simulink model "sm_car_"  (R2026b)
settings: Solver=ode23t  StopTime=100  MaxStep=0.4  AbsTol=1e-3  EnableMultiTasking=on
PreLoadFcn:
  | % Due to usability issue in Repeating Sequence block
  | warning('off','Simulink:Masking:Invalid');
  | 
  | % Eliminate unnecessary warnings in inactive variants
  | % Warnings generated only if you click through inactive variant
  | warning('off','MATLAB:nonExistentField');
  | warning('off','Simulink:Parameters:BlkParamUndefined');
PostLoadFcn:
  | set_param([bdroot '/Vehicle'],'popup_trailer','Off')
  | warning('off','sm:sli:setup:compile:LocalSolverNotSupported')
  | %sm_car_config_maneuver(bdroot,'WOT Braking');
  | sm_car_config_vehicle(bdroot,'false');
  | sm_car_config_logging(bdroot);
InitFcn:
  | sm_car_config_camera;
  | Vehicle = sm_car_vehcfg_checkConfig(Vehicle);
  | sm_car_check_tire_model(bdroot);
StartFcn:
  | tic;
StopFcn:
  | Elapsed_Sim_Time = toc;
  | % disp(['Elapsed Sim Time = ' num2str(Elapsed_Sim_Time)]);
undefined symbols (not defined in the file or in its folder): acc_theta, accel_ramp_rate, Axle1D, AxleIn, Camera, Control, Driver, Init, Maneuver, Pedal, Scene, ShaftL1, ShaftL2, ShaftR1, ShaftR2, Visual, X, xy_data_car_side, Y, Z
libraries: sm_lib x290, fl_lib x171, nesl_utility x144, simulink x60, simulink_extras x14, sdl_lib x14, SimscapeFluids_lib x7, Damper_Element x4, Tire_1x2x x4, ee_lib x3, Scene_Utilities x3, sharedTrackingLibrary x2
(part 12 of 22)

== system sm_car_/Driver/Closed Loop1/Maneuver/PoseTarget Visual/Pace Car ==
  Left Face : sm_lib/Body Elements/Extruded Solid  ExtrusionType=General  PolygonNumSides=3  PolygonOuterRadius=1  PolygonOuterRadiusUnits=m  ExportEntireGeometry=off  ExtrusionCrossSection=xy_data_car_side  ExtrusionCrossSectionUnits=m  ExportConvexHullGeometry=off  ExtrusionLength=thk_side  ExtrusionLengthUnits=m  InertiaType=PointMass  BasedOnType=Density  Density=1000  DensityUnits=kg/m^3  Mass=0  MassUnits=kg  CenterOfMass=[0 0 0]  CenterOfMassUnits=m  MomentsOfInertia=[1 1 1]  MomentsOfInertiaUnits=kg*m^2  ProductsOfInertia=[0 0 0]  ProductsOfInertiaUnits=kg*m^2  GraphicType=FromGeometry  MarkerShape=Sphere  MarkerSize=10  GraphicVisPropType=SimpleVisualProperties  GraphicDiffuseColor=clr_body_geo_left  GraphicOpacity=opc_body_geo_left  GraphicSpecularColor=[0.5 0.5 0.5 1.0]  GraphicAmbientColor=[0.15 0.15 0.15 1.0]  GraphicEmissiveColor=[0.0 0.0 0.0 1.0]  GraphicShininess=75  DoExposeReferenceFrame=on  SerializedFrames=<Frames/>
  Ornament Front : sm_lib/Body Elements/Extruded Solid  ExtrusionType=General  PolygonNumSides=3  PolygonOuterRadius=1  PolygonOuterRadiusUnits=m  ExportEntireGeometry=off  ExtrusionCrossSection=extr_data_emblem_f  ExtrusionCrossSectionUnits=m  ExportConvexHullGeometry=off  ExtrusionLength=0.01  ExtrusionLengthUnits=m  InertiaType=CalculateFromGeometry  BasedOnType=Density  Density=1000  DensityUnits=kg/m^3  Mass=1  MassUnits=kg  CenterOfMass=[0 0 0]  CenterOfMassUnits=m  MomentsOfInertia=[1 1 1]  MomentsOfInertiaUnits=kg*m^2  ProductsOfInertia=[0 0 0]  ProductsOfInertiaUnits=kg*m^2  GraphicType=FromGeometry  MarkerShape=Sphere  MarkerSize=10  GraphicVisPropType=AdvancedVisualProperties  GraphicDiffuseColor=clr_emblem_f  GraphicOpacity=opc_emblem_f  GraphicSpecularColor=[0.5 0.5 0.5 1.0]  GraphicAmbientColor=[0.15 0.15 0.15 1.0]  GraphicEmissiveColor=[clr_emblem_f 1.0]  GraphicShininess=75  DoExposeReferenceFrame=on  SerializedFrames=<Frames/>
  Ornament Rear : sm_lib/Body Elements/Extruded Solid  ExtrusionType=General  PolygonNumSides=3  PolygonOuterRadius=1  PolygonOuterRadiusUnits=m  ExportEntireGeometry=off  ExtrusionCrossSection=extr_data_emblem_r  ExtrusionCrossSectionUnits=m  ExportConvexHullGeometry=off  ExtrusionLength=0.01  ExtrusionLengthUnits=m  InertiaType=CalculateFromGeometry  BasedOnType=Density  Density=1000  DensityUnits=kg/m^3  Mass=1  MassUnits=kg  CenterOfMass=[0 0 0]  CenterOfMassUnits=m  MomentsOfInertia=[1 1 1]  MomentsOfInertiaUnits=kg*m^2  ProductsOfInertia=[0 0 0]  ProductsOfInertiaUnits=kg*m^2  GraphicType=FromGeometry  MarkerShape=Sphere  MarkerSize=10  GraphicVisPropType=SimpleVisualProperties  GraphicDiffuseColor=clr_emblem_r  GraphicOpacity=opc_emblem_r  GraphicSpecularColor=[0.5 0.5 0.5 1.0]  GraphicAmbientColor=[0.15 0.15 0.15 1.0]  GraphicEmissiveColor=[0.0 0.0 0.0 1.0]  GraphicShininess=75  DoExposeReferenceFrame=on  SerializedFrames=<Frames/>
  Rear View : sm_lib/Frames and Transforms/Reference Frame
  Right Face : sm_lib/Body Elements/Extruded Solid  ExtrusionType=General  PolygonNumSides=3  PolygonOuterRadius=1  PolygonOuterRadiusUnits=m  ExportEntireGeometry=off  ExtrusionCrossSection=xy_data_car_side  ExtrusionCrossSectionUnits=m  ExportConvexHullGeometry=off  ExtrusionLength=thk_side  ExtrusionLengthUnits=m  InertiaType=PointMass  BasedOnType=Density  Density=1000  DensityUnits=kg/m^3  Mass=0  MassUnits=kg  CenterOfMass=[0 0 0]  CenterOfMassUnits=m  MomentsOfInertia=[1 1 1]  MomentsOfInertiaUnits=kg*m^2  ProductsOfInertia=[0 0 0]  ProductsOfInertiaUnits=kg*m^2  GraphicType=FromGeometry  MarkerShape=Sphere  MarkerSize=10  GraphicVisPropType=SimpleVisualProperties  GraphicDiffuseColor=clr_body_geo_right  GraphicOpacity=opc_body_geo_right  GraphicSpecularColor=[0.5 0.5 0.5 1.0]  GraphicAmbientColor=[0.15 0.15 0.15 1.0]  GraphicEmissiveColor=[0.0 0.0 0.0 1.0]  GraphicShininess=75  DoExposeReferenceFrame=on  SerializedFrames=<Frames/>
  Top Surface : sm_lib/Body Elements/Extruded Solid  ExtrusionType=General  PolygonNumSides=3  PolygonOuterRadius=1  PolygonOuterRadiusUnits=m  ExportEntireGeometry=off  ExtrusionCrossSection=xy_data_car_top  ExtrusionCrossSectionUnits=m  ExportConvexHullGeometry=off  ExtrusionLength=car_track  ExtrusionLengthUnits=m  InertiaType=PointMass  BasedOnType=Density  Density=0  DensityUnits=kg/m^3  Mass=0  MassUnits=kg  CenterOfMass=[0 0 0]  CenterOfMassUnits=m  MomentsOfInertia=[1 1 1]  MomentsOfInertiaUnits=kg*m^2  ProductsOfInertia=[0 0 0]  ProductsOfInertiaUnits=kg*m^2  GraphicType=FromGeometry  MarkerShape=Sphere  MarkerSize=10  GraphicVisPropType=SimpleVisualProperties  GraphicDiffuseColor=clr_body_geo_top  GraphicOpacity=opc_body_geo_top  GraphicSpecularColor=[0.5 0.5 0.5 1.0]  GraphicAmbientColor=[0.15 0.15 0.15 1.0]  GraphicEmissiveColor=[0.0 0.0 0.0 1.0]  GraphicShininess=75  DoExposeReferenceFrame=on  SerializedFrames=<Frames/>
  Transform Extrusion Axes : sm_lib/Frames and Transforms/Rigid Transform  RotationMethod=StandardAxis  FollAlignAxisA=+X  BaseAlignAxisA=+Y  FollAlignAxisB=+Y  BaseAlignAxisB=+Z  RotationStandardAxis=+X  RotationAngle=90  RotationAngleUnits=deg  RotationArbitraryAxis=[0 0 1]  RotationSequenceAxes=FollowerAxes  RotationSequence=XYX  RotationSequenceAngles=[0 0 0]  RotationSequenceAnglesUnits=deg  RotationMatrix=[1 0 0; 0 1 0; 0 0 1]  Quaternion=[1 0 0 0]  TranslationMethod=None  TranslationCartesianOffset=[0 0 0]  TranslationCartesianOffsetUnits=m  TranslationStandardAxis=+Z  TranslationStandardOffset=0  TranslationStandardOffsetUnits=m  TranslationROffset=0  TranslationROffsetUnits=m  TranslationThetaOffset=0  TranslationThetaOffsetUnits=deg  TranslationZOffset=0  TranslationZOffsetUnits=m
  Transform Ornament Front : sm_lib/Frames and Transforms/Rigid Transform  RotationMethod=RotationSequence  FollAlignAxisA=+X  BaseAlignAxisA=+Y  FollAlignAxisB=+Y  BaseAlignAxisB=+Z  RotationStandardAxis=+Z  RotationAngle=90  RotationAngleUnits=deg  RotationArbitraryAxis=[0 0 1]  RotationSequenceAxes=FollowerAxes  RotationSequence=ZXY  RotationSequenceAngles=[90 90 0]  RotationSequenceAnglesUnits=deg  RotationMatrix=[1 0 0; 0 1 0; 0 0 1]  Quaternion=[1 0 0 0]  TranslationMethod=Cartesian  TranslationCartesianOffset=[max(xy_data_car_side(:,1)) 0 min(xy_data_car_side(:,2))+0.15]  TranslationCartesianOffsetUnits=m  TranslationStandardAxis=+Z  TranslationStandardOffset=1  TranslationStandardOffsetUnits=m  TranslationROffset=0  TranslationROffsetUnits=m  TranslationThetaOffset=0  TranslationThetaOffsetUnits=deg  TranslationZOffset=0  TranslationZOffsetUnits=m
  Transform Ornament Rear : sm_lib/Frames and Transforms/Rigid Transform  RotationMethod=RotationSequence  FollAlignAxisA=+X  BaseAlignAxisA=+Y  FollAlignAxisB=+Y  BaseAlignAxisB=+Z  RotationStandardAxis=+Z  RotationAngle=90  RotationAngleUnits=deg  RotationArbitraryAxis=[0 0 1]  RotationSequenceAxes=FollowerAxes  RotationSequence=ZXY  RotationSequenceAngles=[90 90 180]  RotationSequenceAnglesUnits=deg  RotationMatrix=[1 0 0; 0 1 0; 0 0 1]  Quaternion=[1 0 0 0]  TranslationMethod=Cartesian  TranslationCartesianOffset=[min(xy_data_car_side(:,1))+0.1 0 min(xy_data_car_side(:,2))+0.15]  TranslationCartesianOffsetUnits=m  TranslationStandardAxis=+Z  TranslationStandardOffset=1  TranslationStandardOffsetUnits=m  TranslationROffset=0  TranslationROffsetUnits=m  TranslationThetaOffset=0  TranslationThetaOffsetUnits=deg  TranslationZOffset=0  TranslationZOffsetUnits=m
  Transform Rear View : sm_lib/Frames and Transforms/Rigid Transform  RotationMethod=None  FollAlignAxisA=+X  BaseAlignAxisA=+Y  FollAlignAxisB=+Y  BaseAlignAxisB=+Z  RotationStandardAxis=+Z  RotationAngle=0.0  RotationAngleUnits=deg  RotationArbitraryAxis=[0 0 1]  RotationSequenceAxes=FollowerAxes  RotationSequence=XYX  RotationSequenceAngles=[0 0 0]  RotationSequenceAnglesUnits=deg  RotationMatrix=[1 0 0; 0 1 0; 0 0 1]  Quaternion=[1 0 0 0]  TranslationMethod=Cartesian  TranslationCartesianOffset=[min(xy_data_car_side(:,1))-4 0 min(xy_data_car_side(:,2))+1]  TranslationCartesianOffsetUnits=m  TranslationStandardAxis=+Z  TranslationStandardOffset=0  TranslationStandardOffsetUnits=m  TranslationROffset=0  TranslationROffsetUnits=m  TranslationThetaOffset=0  TranslationThetaOffsetUnits=deg  TranslationZOffset=0  TranslationZOffsetUnits=m
  Transform Reference : sm_lib/Frames and Transforms/Rigid Transform  RotationMethod=None  FollAlignAxisA=+X  BaseAlignAxisA=+Y  FollAlignAxisB=+Y  BaseAlignAxisB=+Z  RotationStandardAxis=+Z  RotationAngle=0.0  RotationAngleUnits=deg  RotationArbitraryAxis=[0 0 1]  RotationSequenceAxes=FollowerAxes  RotationSequence=XYX  RotationSequenceAngles=[0 0 0]  RotationSequenceAnglesUnits=deg  RotationMatrix=[1 0 0; 0 1 0; 0 0 1]  Quaternion=[1 0 0 0]  TranslationMethod=Cartesian  TranslationCartesianOffset=offset_ref  TranslationCartesianOffsetUnits=m  TranslationStandardAxis=+Z  TranslationStandardOffset=0  TranslationStandardOffsetUnits=m  TranslationROffset=0  TranslationROffsetUnits=m  TranslationThetaOffset=0  TranslationThetaOffsetUnits=deg  TranslationZOffset=0  TranslationZOffsetUnits=m
  Transform Left Face : sm_lib/Frames and Transforms/Rigid Transform  RotationMethod=None  FollAlignAxisA=+X  BaseAlignAxisA=+Y  FollAlignAxisB=+Y  BaseAlignAxisB=+Z  RotationStandardAxis=+Z  RotationAngle=0.0  RotationAngleUnits=deg  RotationArbitraryAxis=[0 0 1]  RotationSequenceAxes=FollowerAxes  RotationSequence=XYX  RotationSequenceAngles=[0 0 0]  RotationSequenceAnglesUnits=deg  RotationMatrix=[1 0 0; 0 1 0; 0 0 1]  Quaternion=[1 0 0 0]  TranslationMethod=StandardAxis  TranslationCartesianOffset=[0 0 0]  TranslationCartesianOffsetUnits=m  TranslationStandardAxis=-Z  TranslationStandardOffset=car_track/2-thk_side/2  TranslationStandardOffsetUnits=m  TranslationROffset=0  TranslationROffsetUnits=m  TranslationThetaOffset=0  TranslationThetaOffsetUnits=deg  TranslationZOffset=0  TranslationZOffsetUnits=m
  Transform Right Face : sm_lib/Frames and Transforms/Rigid Transform  RotationMethod=None  FollAlignAxisA=+X  BaseAlignAxisA=+Y  FollAlignAxisB=+Y  BaseAlignAxisB=+Z  RotationStandardAxis=+Z  RotationAngle=0.0  RotationAngleUnits=deg  RotationArbitraryAxis=[0 0 1]  RotationSequenceAxes=FollowerAxes  RotationSequence=XYX  RotationSequenceAngles=[0 0 0]  RotationSequenceAnglesUnits=deg  RotationMatrix=[1 0 0; 0 1 0; 0 0 1]  Quaternion=[1 0 0 0]  TranslationMethod=StandardAxis  TranslationCartesianOffset=[0 0 0]  TranslationCartesianOffsetUnits=m  TranslationStandardAxis=+Z  TranslationStandardOffset=car_track/2-thk_side/2  TranslationStandardOffsetUnits=m  TranslationROffset=0  TranslationROffsetUnits=m  TranslationThetaOffset=0  TranslationThetaOffsetUnits=deg  TranslationZOffset=0  TranslationZOffsetUnits=m
  FA : PMIOPort  Side=Right
  P : PMIOPort  Port=2  Side=Left
  connections:
  Transform Reference/LConn1 -- P/RConn1 -- FA/RConn1
  Transform Rear View/RConn1 -- Rear View/RConn1
  Transform Reference/RConn1 -- Transform Ornament Front/LConn1 -- Transform Ornament Rear/LConn1 -- Transform Rear View/LConn1 -- Transform Extrusion Axes/LConn1
  Left Face/RConn1 -- Transform Left Face/RConn1
  Transform Extrusion Axes/RConn1 -- Transform Right Face/LConn1 -- Top Surface/RConn1 -- Transform Left Face/LConn1
  Right Face/RConn1 -- Transform Right Face/RConn1
  Transform Ornament Front/RConn1 -- Ornament Front/RConn1
  Transform Ornament Rear/RConn1 -- Ornament Rear/RConn1

== system sm_car_/Vehicle/Vehicle/Brakes/PedalAbstract DiscDisc/Actuator L1 ==
  Pedal : Inport
  Filter : TransferFcn  Numerator=brk_max_p  Denominator=[brk_filt 1]
  Simulink-PS Converter : nesl_utility/Simulink-PS Converter  PhysicalDomain=network_engine_domain  SubClassName=ps_input  LeftPortType=input  RightPortType=output  PseudoPeriodic=off  Frequencies=[]  NoiseDistribution=none  NoiseParameters=[]  Unit=1  AffineConversion=off  FilteringAndDerivatives=provide  SimscapeFilterOrder=1  InputFilterTimeConstant=0.001  UdotUserProvided=0
  P : PMIOPort  Side=Right
  wires:
  Pedal/1 -> Filter/1
  Filter/1 -> Simulink-PS Converter/1
  connections:
  Simulink-PS Converter/RConn1 -- P/RConn1

== system sm_car_/Vehicle/Vehicle/Brakes/PedalAbstract DiscDisc/Actuator L2 ==
  Pedal : Inport
  Filter : TransferFcn  Numerator=brk_max_p  Denominator=[brk_filt 1]
  Simulink-PS Converter : nesl_utility/Simulink-PS Converter  PhysicalDomain=network_engine_domain  SubClassName=ps_input  LeftPortType=input  RightPortType=output  PseudoPeriodic=off  Frequencies=[]  NoiseDistribution=none  NoiseParameters=[]  Unit=1  AffineConversion=off  FilteringAndDerivatives=provide  SimscapeFilterOrder=1  InputFilterTimeConstant=0.001  UdotUserProvided=0
  P : PMIOPort  Side=Right
  wires:
  Pedal/1 -> Filter/1
  Filter/1 -> Simulink-PS Converter/1
  connections:
  Simulink-PS Converter/RConn1 -- P/RConn1

== system sm_car_/Vehicle/Vehicle/Brakes/PedalAbstract DiscDisc/Actuator R1 ==
  Pedal : Inport
  Filter : TransferFcn  Numerator=brk_max_p  Denominator=[brk_filt 1]
  Simulink-PS Converter : nesl_utility/Simulink-PS Converter  PhysicalDomain=network_engine_domain  SubClassName=ps_input  LeftPortType=input  RightPortType=output  PseudoPeriodic=off  Frequencies=[]  NoiseDistribution=none  NoiseParameters=[]  Unit=1  AffineConversion=off  FilteringAndDerivatives=provide  SimscapeFilterOrder=1  InputFilterTimeConstant=0.001  UdotUserProvided=0
  P : PMIOPort  Side=Right
  wires:
  Pedal/1 -> Filter/1
  Filter/1 -> Simulink-PS Converter/1
  connections:
  Simulink-PS Converter/RConn1 -- P/RConn1

== system sm_car_/Vehicle/Vehicle/Brakes/PedalAbstract DiscDisc/Actuator R2 ==
  Pedal : Inport
  Filter : TransferFcn  Numerator=brk_max_p  Denominator=[brk_filt 1]
  Simulink-PS Converter : nesl_utility/Simulink-PS Converter  PhysicalDomain=network_engine_domain  SubClassName=ps_input  LeftPortType=input  RightPortType=output  PseudoPeriodic=off  Frequencies=[]  NoiseDistribution=none  NoiseParameters=[]  Unit=1  AffineConversion=off  FilteringAndDerivatives=provide  SimscapeFilterOrder=1  InputFilterTimeConstant=0.001  UdotUserProvided=0
  P : PMIOPort  Side=Right
  wires:
  Pedal/1 -> Filter/1
  Filter/1 -> Simulink-PS Converter/1
  connections:
  Simulink-PS Converter/RConn1 -- P/RConn1

== system sm_car_/Vehicle/Vehicle/Brakes/PedalAbstract DiscDisc/Sensing Torque L1 ==
  Ideal Torque Sensor : fl_lib/Mechanical/Mechanical Sensors/Ideal Torque Sensor
  PS-Simulink Converter : nesl_utility/PS-Simulink Converter  PhysicalDomain=network_engine_domain  SubClassName=ps_output  LeftPortType=input  RightPortType=output  PseudoPeriodic=off  Frequencies=[]  VectorFormat=1-D array  Unit=N*m  AffineConversion=off
  C : PMIOPort  Side=Right
  R : PMIOPort  Port=2  Side=Left
  T : Outport  VectorParamsAs1DForOutWhenUnconnected=off
  wires:
  PS-Simulink Converter/1 -> T/1
  connections:
  PS-Simulink Converter/LConn1 -- Ideal Torque Sensor/RConn2
  Ideal Torque Sensor/RConn1 -- C/RConn1
  Ideal Torque Sensor/LConn1 -- R/RConn1

== system sm_car_/Vehicle/Vehicle/Brakes/PedalAbstract DiscDisc/Sensing Torque L2 ==
  Ideal Torque Sensor : fl_lib/Mechanical/Mechanical Sensors/Ideal Torque Sensor
  PS-Simulink Converter : nesl_utility/PS-Simulink Converter  PhysicalDomain=network_engine_domain  SubClassName=ps_output  LeftPortType=input  RightPortType=output  PseudoPeriodic=off  Frequencies=[]  VectorFormat=1-D array  Unit=N*m  AffineConversion=off
  C : PMIOPort  Side=Right
  R : PMIOPort  Port=2  Side=Left
  T : Outport  VectorParamsAs1DForOutWhenUnconnected=off
  wires:
  PS-Simulink Converter/1 -> T/1
  connections:
  PS-Simulink Converter/LConn1 -- Ideal Torque Sensor/RConn2
  Ideal Torque Sensor/RConn1 -- C/RConn1
  Ideal Torque Sensor/LConn1 -- R/RConn1

== system sm_car_/Vehicle/Vehicle/Brakes/PedalAbstract DiscDisc/Sensing Torque R1 ==
  Ideal Torque Sensor : fl_lib/Mechanical/Mechanical Sensors/Ideal Torque Sensor
  PS-Simulink Converter : nesl_utility/PS-Simulink Converter  PhysicalDomain=network_engine_domain  SubClassName=ps_output  LeftPortType=input  RightPortType=output  PseudoPeriodic=off  Frequencies=[]  VectorFormat=1-D array  Unit=N*m  AffineConversion=off
  C : PMIOPort  Side=Right
  R : PMIOPort  Port=2  Side=Left
  T : Outport  VectorParamsAs1DForOutWhenUnconnected=off
  wires:
  PS-Simulink Converter/1 -> T/1
  connections:
  Ideal Torque Sensor/LConn1 -- R/RConn1
  Ideal Torque Sensor/RConn1 -- C/RConn1
  PS-Simulink Converter/LConn1 -- Ideal Torque Sensor/RConn2

== system sm_car_/Vehicle/Vehicle/Brakes/PedalAbstract DiscDisc/Sensing Torque R2 ==
  Ideal Torque Sensor : fl_lib/Mechanical/Mechanical Sensors/Ideal Torque Sensor
  PS-Simulink Converter : nesl_utility/PS-Simulink Converter  PhysicalDomain=network_engine_domain  SubClassName=ps_output  LeftPortType=input  RightPortType=output  PseudoPeriodic=off  Frequencies=[]  VectorFormat=1-D array  Unit=N*m  AffineConversion=off
  C : PMIOPort  Side=Right
  R : PMIOPort  Port=2  Side=Left
  T : Outport  VectorParamsAs1DForOutWhenUnconnected=off
  wires:
  PS-Simulink Converter/1 -> T/1
  connections:
  Ideal Torque Sensor/LConn1 -- R/RConn1
  Ideal Torque Sensor/RConn1 -- C/RConn1
  PS-Simulink Converter/LConn1 -- Ideal Torque Sensor/RConn2

== system sm_car_/Vehicle/Vehicle/Chassis/Aero/Subsystem ==
  RdBus : Inport
  Actuator dynamics : Subsystem  mask(First-order lag supporting vector signals){b=0.5, x_initial=0}
      mask prompts: b "Filter time constant"; x_initial "Initial output"
      mask help: Models a lag of the form 1/(b*s+1) where s is the Laplace operator.
  Bus Selector : BusSelector  OutputSignals=fx,fy,fz
  Mux : Mux  Inputs=3
  Simulink-PS Converter : nesl_utility/Simulink-PS Converter  PhysicalDomain=network_engine_domain  SubClassName=ps_input  LeftPortType=input  RightPortType=output  PseudoPeriodic=off  Frequencies=[]  NoiseDistribution=none  NoiseParameters=[]  Unit=1  AffineConversion=off  FilteringAndDerivatives=provide  SimscapeFilterOrder=1  InputFilterTimeConstant=0.001  UdotUserProvided=0
  fWind : PMIOPort  Side=Right
  wires:
  Actuator dynamics/1(Out) -> Simulink-PS Converter/1
  RdBus/1 -> Bus Selector/1
  Bus Selector/3 -> Mux/3  "<fz>"
  Bus Selector/2 -> Mux/2  "<fy>"
  Bus Selector/1 -> Mux/1  "<fx>"
  Mux/1 -> Actuator dynamics/1(In)
  connections:
  Simulink-PS Converter/RConn1 -- fWind/RConn1

== system sm_car_/Vehicle/Vehicle/Chassis/Body/Body Geometry ==
  CAD FSAE Achilles : Subsystem  VariantControl=CAD_FSAE_Achilles  mask(FSAE Body Geometry){body_offset=BodyGeometry.sOffset.Value, body_orient=BodyGeometry.aOffset.Value, body_clr=BodyGeometry.Color.Value, body_opc=BodyGeometry.Opacity.Value, aero_clr=BodyGeometry.AeroColor.Value, aero_opc=BodyGeometry.AeroOpacity.Value, extr_data_emblem_aero=Visual.PaceCar.emblem.data*0.3, extr_data_emblem_hood=Visual.PaceCar.emblem.data*0.3, clr_emblem_aero=Visual.clr.orange, clr_emblem_hood=Visual.clr.orange, opc_emblem_aero=Visual.emblem.opc, opc_emblem_hood=Visual.emblem.opc}
      mask prompts: body_offset "Body Offset [x y z] (m)"; body_orient "Body Orientation [R P Y] (rad)"; body_clr "Body Color [R G B] (0-1)"; body_opc "Body Opacity (0-1)"; aero_clr "Aero Color [R G B] (0-1)"; aero_opc "Aero Opacity (0-1)"; extr_data_emblem_aero "Emblem Data Aero [xy] (m)"; extr_data_emblem_hood "Emblem Data Hood [xy] (m)"; clr_emblem_aero "Emblem Color Aero [R G B] (0-1)"; clr_emblem_hood "Emblem Color Hood [R G B] (0-1)"; opc_emblem_aero "Emblem Opacity Aero (0-1)"; opc_emblem_hood "Emblem Opacity Hood (0-1)"
      mask help: CAD geometry of Formula Student Vehicle.
      mask TypeOptions extr_data_emblem_aero:
      | Aero/Ornament
      | Left/ExtrusionCrossSection | Aero/Ornament
      | Right/ExtrusionCrossSection
      mask TypeOptions extr_data_emblem_hood:
      | Body/Ornament
      | Hood/ExtrusionCrossSection
      mask TypeOptions clr_emblem_aero:
      | Aero/Ornament
      | Left/GraphicDiffuseColor | Aero/Ornament
      | Right/GraphicDiffuseColor
      mask TypeOptions clr_emblem_hood:
      | Body/Ornament
      | Hood/GraphicDiffuseColor
      mask TypeOptions opc_emblem_aero:
      | Aero/Ornament
      | Left/GraphicOpacity | Aero/Ornament
      | Right/GraphicOpacity
      mask TypeOptions opc_emblem_hood:
      | Body/Ornament
      | Hood/GraphicOpacity
      mask DialogControl cont_emblem Prompt: Emblem
      mask Display: image('sm_car_bodygeometry_cad_fsae_achilles.png');
  FA : PMIOPort  Side=Right
  P : PMIOPort  Port=2  Side=Left

== system sm_car_/Vehicle/Vehicle/Chassis/Body/Body Load ==
  None : Subsystem  VariantControl=None
  " FA" : PMIOPort  Side=Left

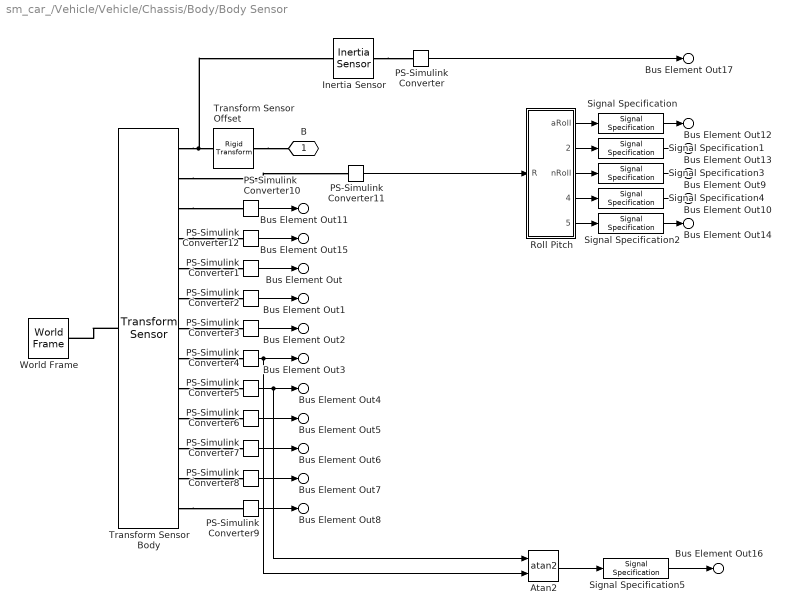
== system sm_car_/Vehicle/Vehicle/Chassis/Body/Body Sensor ==
  Atan2 : Trigonometry  Operator=atan2
  Inertia Sensor : sm_lib/Body Elements/Inertia Sensor  SensorExtent=Mechanism  SpanWeldJoints=off  ExcludeGroundedBodies=on  MeasurementFrame=Attached  SenseMass=off  SenseCenterOfMass=off  SenseInertiaMatrix=off  SenseCenteredInertiaMatrix=on  SensePrincipalInertiaMatrix=off  SenseRotationMatrix=off  GraphicType=PrincipalInertiaFrame  PrincipalInertiaFrameSize=20  GraphicVisPropType=SimpleVisualProperties  GraphicDiffuseColor=[0.5 0.5 0.5]  GraphicOpacity=1  GraphicSpecularColor=[0.5 0.5 0.5 1.0]  GraphicAmbientColor=[0.15 0.15 0.15 1.0]  GraphicEmissiveColor=[0.0 0.0 0.0 1.0]  GraphicShininess=75
  PS-Simulink Converter : nesl_utility/PS-Simulink Converter  PhysicalDomain=network_engine_domain  SubClassName=ps_output  LeftPortType=input  RightPortType=output  PseudoPeriodic=off  Frequencies=[]  VectorFormat=inherit  Unit=kg*m^2  AffineConversion=off
  PS-Simulink Converter1 : nesl_utility/PS-Simulink Converter  PhysicalDomain=network_engine_domain  SubClassName=ps_output  LeftPortType=input  RightPortType=output  PseudoPeriodic=off  Frequencies=[]  VectorFormat=1-D array  Unit=m  AffineConversion=off
  PS-Simulink Converter10 : nesl_utility/PS-Simulink Converter  PhysicalDomain=network_engine_domain  SubClassName=ps_output  LeftPortType=input  RightPortType=output  PseudoPeriodic=off  Frequencies=[]  VectorFormat=inherit  Unit=rad/s  AffineConversion=off
  PS-Simulink Converter11 : nesl_utility/PS-Simulink Converter  PhysicalDomain=network_engine_domain  SubClassName=ps_output  LeftPortType=input  RightPortType=output  PseudoPeriodic=off  Frequencies=[]  VectorFormat=1-D array  Unit=1  AffineConversion=off
  PS-Simulink Converter12 : nesl_utility/PS-Simulink Converter  PhysicalDomain=network_engine_domain  SubClassName=ps_output  LeftPortType=input  RightPortType=output  PseudoPeriodic=off  Frequencies=[]  VectorFormat=inherit  Unit=rad/s^2  AffineConversion=off
  PS-Simulink Converter2 : nesl_utility/PS-Simulink Converter  PhysicalDomain=network_engine_domain  SubClassName=ps_output  LeftPortType=input  RightPortType=output  PseudoPeriodic=off  Frequencies=[]  VectorFormat=1-D array  Unit=m  AffineConversion=off
  PS-Simulink Converter3 : nesl_utility/PS-Simulink Converter  PhysicalDomain=network_engine_domain  SubClassName=ps_output  LeftPortType=input  RightPortType=output  PseudoPeriodic=off  Frequencies=[]  VectorFormat=1-D array  Unit=m  AffineConversion=off
  PS-Simulink Converter4 : nesl_utility/PS-Simulink Converter  PhysicalDomain=network_engine_domain  SubClassName=ps_output  LeftPortType=input  RightPortType=output  PseudoPeriodic=off  Frequencies=[]  VectorFormat=1-D array  Unit=m/s  AffineConversion=off
  PS-Simulink Converter5 : nesl_utility/PS-Simulink Converter  PhysicalDomain=network_engine_domain  SubClassName=ps_output  LeftPortType=input  RightPortType=output  PseudoPeriodic=off  Frequencies=[]  VectorFormat=1-D array  Unit=m/s  AffineConversion=off
  PS-Simulink Converter6 : nesl_utility/PS-Simulink Converter  PhysicalDomain=network_engine_domain  SubClassName=ps_output  LeftPortType=input  RightPortType=output  PseudoPeriodic=off  Frequencies=[]  VectorFormat=1-D array  Unit=m/s  AffineConversion=off
  PS-Simulink Converter7 : nesl_utility/PS-Simulink Converter  PhysicalDomain=network_engine_domain  SubClassName=ps_output  LeftPortType=input  RightPortType=output  PseudoPeriodic=off  Frequencies=[]  VectorFormat=1-D array  Unit=m/s^2  AffineConversion=off
  PS-Simulink Converter8 : nesl_utility/PS-Simulink Converter  PhysicalDomain=network_engine_domain  SubClassName=ps_output  LeftPortType=input  RightPortType=output  PseudoPeriodic=off  Frequencies=[]  VectorFormat=1-D array  Unit=m/s^2  AffineConversion=off
  PS-Simulink Converter9 : nesl_utility/PS-Simulink Converter  PhysicalDomain=network_engine_domain  SubClassName=ps_output  LeftPortType=input  RightPortType=output  PseudoPeriodic=off  Frequencies=[]  VectorFormat=1-D array  Unit=m/s^2  AffineConversion=off
  Roll Pitch : Subsystem
  Signal Specification{,1..2,5} (4 alike) : SignalSpecification  Unit=rad
  Signal Specification3 : SignalSpecification  Unit=rad/s
  Signal Specification4 : SignalSpecification  Unit=rad/s
  Transform Sensor Offset : sm_lib/Frames and Transforms/Rigid Transform  RotationMethod=None  FollAlignAxisA=+X  BaseAlignAxisA=+Y  FollAlignAxisB=+Y  BaseAlignAxisB=+Z  RotationStandardAxis=+Z  RotationAngle=0.0  RotationAngleUnits=deg  RotationArbitraryAxis=[0 0 1]  RotationSequenceAxes=FollowerAxes  RotationSequence=XYX  RotationSequenceAngles=[0 0 0]  RotationSequenceAnglesUnits=deg  RotationMatrix=[1 0 0; 0 1 0; 0 0 1]  Quaternion=[1 0 0 0]  TranslationMethod=Cartesian  TranslationCartesianOffset=offset_body_sensor  TranslationCartesianOffsetUnits=m  TranslationStandardAxis=+Z  TranslationStandardOffset=0  TranslationStandardOffsetUnits=m  TranslationROffset=0  TranslationROffsetUnits=m  TranslationThetaOffset=0  TranslationThetaOffsetUnits=deg  TranslationZOffset=0  TranslationZOffsetUnits=m
  Transform Sensor Body : sm_lib/Frames and Transforms/Transform Sensor  ObservationFrame=World  ExpressedInFrame=Follower  RotationSequence=XYX  SenseAngle=off  SenseAxis=off  SenseQ=off  SenseR=on  SenseRotationSequence=off  SenseOmegaX=off  SenseOmegaY=off  SenseOmegaZ=on  SenseOmega=off  SenseQDot=off  SenseRDot=off  SenseRotationSequenceDot=off  SenseAlphaX=off  SenseAlphaY=off  SenseAlphaZ=on  SenseAlpha=off  SenseQDDot=off  SenseRDDot=off  SenseX=on  SenseY=on  SenseZ=on  SenseXYZ=off  SenseRad=off  SenseAzim=off  SenseDist=off  SenseInc=off  SenseXDot=on  SenseYDot=on  SenseZDot=on  SenseXYZDot=off  SenseRadDot=off  SenseAzimDot=off  SenseDistDot=off  SenseIncDot=off  SenseXDDot=on  SenseYDDot=on  SenseZDDot=on  SenseXYZDDot=off  SenseRadDDot=off  SenseAzimDDot=off  SenseDistDDot=off  SenseIncDDot=off
  World Frame : sm_lib/Frames and Transforms/World Frame
  B : PMIOPort  Side=Left
  Bus Element Out : Outport  VectorParamsAs1DForOutWhenUnconnected=off  PortName=Body  Element=x
  Bus Element Out1 : Outport  VectorParamsAs1DForOutWhenUnconnected=off  PortName=Body  Element=y
  Bus Element Out2 : Outport  VectorParamsAs1DForOutWhenUnconnected=off  PortName=Body  Element=z
  Bus Element Out3 : Outport  VectorParamsAs1DForOutWhenUnconnected=off  PortName=Body  Element=vx
  Bus Element Out4 : Outport  VectorParamsAs1DForOutWhenUnconnected=off  PortName=Body  Element=vy
  Bus Element Out5 : Outport  VectorParamsAs1DForOutWhenUnconnected=off  PortName=Body  Element=vz
  Bus Element Out6 : Outport  VectorParamsAs1DForOutWhenUnconnected=off  PortName=Body  Element=gx
  Bus Element Out7 : Outport  VectorParamsAs1DForOutWhenUnconnected=off  PortName=Body  Element=gy
  Bus Element Out8 : Outport  VectorParamsAs1DForOutWhenUnconnected=off  PortName=Body  Element=gz
  Bus Element Out9 : Outport  VectorParamsAs1DForOutWhenUnconnected=off  PortName=Body  Element=nRoll
  Bus Element Out10 : Outport  VectorParamsAs1DForOutWhenUnconnected=off  PortName=Body  Element=nPitch
  Bus Element Out11 : Outport  VectorParamsAs1DForOutWhenUnconnected=off  PortName=Body  Element=nYaw
  Bus Element Out12 : Outport  VectorParamsAs1DForOutWhenUnconnected=off  PortName=Body  Element=aRoll
  Bus Element Out13 : Outport  VectorParamsAs1DForOutWhenUnconnected=off  PortName=Body  Element=aPitch
  Bus Element Out14 : Outport  VectorParamsAs1DForOutWhenUnconnected=off  PortName=Body  Element=aYaw
  Bus Element Out15 : Outport  VectorParamsAs1DForOutWhenUnconnected=off  PortName=Body  Element=gYaw
  Bus Element Out16 : Outport  VectorParamsAs1DForOutWhenUnconnected=off  PortName=Body  Element=aSideSlip
  Bus Element Out17 : Outport  VectorParamsAs1DForOutWhenUnconnected=off  PortName=Body  Element=InertiaMatrix
  wires:
  PS-Simulink Converter9/1 -> Bus Element Out8/1
  PS-Simulink Converter11/1 -> Roll Pitch/1(R)
  PS-Simulink Converter6/1 -> Bus Element Out5/1
  PS-Simulink Converter7/1 -> Bus Element Out6/1
  PS-Simulink Converter2/1 -> Bus Element Out1/1
  PS-Simulink Converter8/1 -> Bus Element Out7/1
  PS-Simulink Converter5/1 -> Atan2/1, Bus Element Out4/1
  PS-Simulink Converter3/1 -> Bus Element Out2/1
  PS-Simulink Converter1/1 -> Bus Element Out/1
  PS-Simulink Converter4/1 -> Bus Element Out3/1, Atan2/2
  Signal Specification/1 -> Bus Element Out12/1
  Signal Specification1/1 -> Bus Element Out13/1
  Signal Specification2/1 -> Bus Element Out14/1
  Signal Specification3/1 -> Bus Element Out9/1
  Signal Specification4/1 -> Bus Element Out10/1
  Roll Pitch/5(aYaw) -> Signal Specification2/1
  Roll Pitch/3(nRoll) -> Signal Specification3/1
  Roll Pitch/4(nPitch) -> Signal Specification4/1
  Roll Pitch/2(aPitch) -> Signal Specification1/1
  Roll Pitch/1(aRoll) -> Signal Specification/1
  PS-Simulink Converter/1 -> Bus Element Out17/1
  PS-Simulink Converter10/1 -> Bus Element Out11/1
  PS-Simulink Converter12/1 -> Bus Element Out15/1
  Signal Specification5/1 -> Bus Element Out16/1
  Atan2/1 -> Signal Specification5/1
  connections:
  Transform Sensor Body/RConn2 -- PS-Simulink Converter11/LConn1
  Transform Sensor Body/LConn1 -- World Frame/RConn1
  Transform Sensor Offset/LConn1 -- B/RConn1
  Transform Sensor Body/RConn1 -- Inertia Sensor/LConn1 -- Transform Sensor Offset/RConn1
  Inertia Sensor/RConn1 -- PS-Simulink Converter/LConn1
  Transform Sensor Body/RConn5 -- PS-Simulink Converter1/LConn1
  Transform Sensor Body/RConn6 -- PS-Simulink Converter2/LConn1
  Transform Sensor Body/RConn7 -- PS-Simulink Converter3/LConn1
  Transform Sensor Body/RConn8 -- PS-Simulink Converter4/LConn1
  Transform Sensor Body/RConn9 -- PS-Simulink Converter5/LConn1
  Transform Sensor Body/RConn10 -- PS-Simulink Converter6/LConn1
  Transform Sensor Body/RConn11 -- PS-Simulink Converter7/LConn1
  Transform Sensor Body/RConn12 -- PS-Simulink Converter8/LConn1
  Transform Sensor Body/RConn13 -- PS-Simulink Converter9/LConn1
  Transform Sensor Body/RConn3 -- PS-Simulink Converter10/LConn1
  Transform Sensor Body/RConn4 -- PS-Simulink Converter12/LConn1

== system sm_car_/Vehicle/Vehicle/Chassis/Damper/Decoupled ==
  In Bus Element1 : Inport  PortName=Ctrl  Element=L1
  In Bus Element : Inport  PortName=Ctrl  Element=R1
  In Bus Element2 : Inport  PortName=Ctrl  Element=L2
  In Bus Element3 : Inport  PortName=Ctrl  Element=R2
  Damper A1 Heave : Subsystem  Variant=on  VariantControlMode=label  VariantControl=Variant1  LabelModeActiveChoice=Linear  mask(Variants for Damper){Damper=Damper.Axle1.Heave, VariantLabel=Damper.Axle1.Heave.class.Value}
      mask prompts: Damper "Damper Parameters"; VariantLabel "Variant Label"
      mask help: Select option and provide parameters for damper. Option is chosen by string provided in Variant Label. The parameters for the selected option is contained in Damper data structure.
      mask init:
      | curblk = gcb;
      | 
      | % Set variant for this block 
      | set_param(curblk,'LabelModeActiveChoice',VariantLabel);
      settings: AttributesFormatString=%<ActiveVariant>
      mask Display: disp(' ')
  Damper A1 Roll : Subsystem  Variant=on  VariantControlMode=label  VariantControl=Variant1  LabelModeActiveChoice=Linear  mask(Variants for Damper){Damper=Damper.Axle1.Roll, VariantLabel=Damper.Axle1.Roll.class.Value}
      mask prompts: Damper "Damper Parameters"; VariantLabel "Variant Label"
      mask help: Select option and provide parameters for damper. Option is chosen by string provided in Variant Label. The parameters for the selected option is contained in Damper data structure.
      mask init:
      | curblk = gcb;
      | 
      | % Set variant for this block 
      | set_param(curblk,'LabelModeActiveChoice',VariantLabel);
      settings: AttributesFormatString=%<ActiveVariant>
      mask Display: disp(' ')
  Damper A2 Heave : Subsystem  Variant=on  VariantControlMode=label  VariantControl=Variant1  LabelModeActiveChoice=Linear  mask(Variants for Damper){Damper=Damper.Axle2.Heave, VariantLabel=Damper.Axle2.Heave.class.Value}
      mask prompts: Damper "Damper Parameters"; VariantLabel "Variant Label"
      mask help: Select option and provide parameters for damper. Option is chosen by string provided in Variant Label. The parameters for the selected option is contained in Damper data structure.
      mask init:
      | curblk = gcb;
      | 
      | % Set variant for this block 
      | set_param(curblk,'LabelModeActiveChoice',VariantLabel);
      settings: AttributesFormatString=%<ActiveVariant>
      mask Display: disp(' ')
  Damper A2 Roll : Subsystem  Variant=on  VariantControlMode=label  VariantControl=Variant1  LabelModeActiveChoice=Linear  mask(Variants for Damper){Damper=Damper.Axle2.Roll, VariantLabel=Damper.Axle2.Roll.class.Value}
      mask prompts: Damper "Damper Parameters"; VariantLabel "Variant Label"
      mask help: Select option and provide parameters for damper. Option is chosen by string provided in Variant Label. The parameters for the selected option is contained in Damper data structure.
      mask init:
      | curblk = gcb;
      | 
      | % Set variant for this block 
      | set_param(curblk,'LabelModeActiveChoice',VariantLabel);
      settings: AttributesFormatString=%<ActiveVariant>
      mask Display: disp(' ')
  MTRef L1 : fl_lib/Mechanical/Translational Elements/Mechanical Translational Reference
  MTRef L2 : fl_lib/Mechanical/Translational Elements/Mechanical Translational Reference
  MTRef R1 : fl_lib/Mechanical/Translational Elements/Mechanical Translational Reference
  MTRef R2 : fl_lib/Mechanical/Translational Elements/Mechanical Translational Reference
  L1 : PMIOPort  Side=Left
  R1 : PMIOPort  Port=2  Side=Right
  L2 : PMIOPort  Port=3  Side=Left
  R2 : PMIOPort  Port=4  Side=Right
  Out Bus Element : Outport  VectorParamsAs1DForOutWhenUnconnected=off  PortName=meas  Element=L1
  Out Bus Element1 : Outport  VectorParamsAs1DForOutWhenUnconnected=off  PortName=meas  Element=R1
  Out Bus Element2 : Outport  VectorParamsAs1DForOutWhenUnconnected=off  PortName=meas  Element=L2
  Out Bus Element3 : Outport  VectorParamsAs1DForOutWhenUnconnected=off  PortName=meas  Element=R2
  wires:
  In Bus Element/1 -> Damper A1 Roll/1("Ctrl ")
  In Bus Element1/1 -> Damper A1 Heave/1("Ctrl ")
  Damper A1 Heave/1(" meas") -> Out Bus Element/1
  Damper A1 Roll/1(" meas") -> Out Bus Element1/1
  In Bus Element3/1 -> Damper A2 Roll/1("Ctrl ")
  In Bus Element2/1 -> Damper A2 Heave/1("Ctrl ")
  Damper A2 Heave/1(" meas") -> Out Bus Element2/1
  Damper A2 Roll/1(" meas") -> Out Bus Element3/1
  connections:
  Damper A1 Roll/LConn1 -- R1/RConn1
  Damper A1 Roll/RConn1 -- MTRef R1/LConn1
  Damper A2 Roll/LConn1 -- R2/RConn1
  Damper A2 Roll/RConn1 -- MTRef R2/LConn1
  Damper A2 Heave/LConn1 -- L2/RConn1
  Damper A2 Heave/RConn1 -- MTRef L2/LConn1
  Damper A1 Heave/LConn1 -- L1/RConn1
  Damper A1 Heave/RConn1 -- MTRef L1/LConn1

== system sm_car_/Vehicle/Vehicle/Chassis/Damper/Independent ==
  In Bus Element1 : Inport  PortName=Ctrl  Element=L1
  In Bus Element : Inport  PortName=Ctrl  Element=R1
  In Bus Element2 : Inport  PortName=Ctrl  Element=L2
  In Bus Element3 : Inport  PortName=Ctrl  Element=R2
  Damper : Damper_Element/Damper  VariantControl=Variant1  LabelModeActiveChoice=Nonlinear  Damper=Damper.Axle1  VariantLabel=Damper.Axle1.class.Value
      settings: AttributesFormatString=%<ActiveVariant>
  Damper1 : Damper_Element/Damper  VariantControl=Variant1  LabelModeActiveChoice=Nonlinear  Damper=Damper.Axle1  VariantLabel=Damper.Axle1.class.Value
      settings: AttributesFormatString=%<ActiveVariant>
  Damper2 : Damper_Element/Damper  VariantControl=Variant1  LabelModeActiveChoice=Nonlinear  Damper=Damper.Axle2  VariantLabel=Damper.Axle2.class.Value
      settings: AttributesFormatString=%<ActiveVariant>
  Damper3 : Damper_Element/Damper  VariantControl=Variant1  LabelModeActiveChoice=Nonlinear  Damper=Damper.Axle2  VariantLabel=Damper.Axle2.class.Value
      settings: AttributesFormatString=%<ActiveVariant>
  MTRef L1 : fl_lib/Mechanical/Translational Elements/Mechanical Translational Reference
  MTRef L2 : fl_lib/Mechanical/Translational Elements/Mechanical Translational Reference
  MTRef R1 : fl_lib/Mechanical/Translational Elements/Mechanical Translational Reference
  MTRef R2 : fl_lib/Mechanical/Translational Elements/Mechanical Translational Reference
  L1 : PMIOPort  Side=Left
  R1 : PMIOPort  Port=2  Side=Right
  L2 : PMIOPort  Port=3  Side=Left
  R2 : PMIOPort  Port=4  Side=Right
  Out Bus Element : Outport  VectorParamsAs1DForOutWhenUnconnected=off  PortName=meas  Element=L1
  Out Bus Element1 : Outport  VectorParamsAs1DForOutWhenUnconnected=off  PortName=meas  Element=R1
  Out Bus Element2 : Outport  VectorParamsAs1DForOutWhenUnconnected=off  PortName=meas  Element=L2
  Out Bus Element3 : Outport  VectorParamsAs1DForOutWhenUnconnected=off  PortName=meas  Element=R2
  wires:
  In Bus Element/1 -> Damper1/1
  In Bus Element1/1 -> Damper/1
  Damper/1 -> Out Bus Element/1
  Damper1/1 -> Out Bus Element1/1
  In Bus Element3/1 -> Damper2/1
  In Bus Element2/1 -> Damper3/1
  Damper3/1 -> Out Bus Element2/1
  Damper2/1 -> Out Bus Element3/1
  connections:
  Damper1/LConn1 -- R1/RConn1
  Damper1/RConn1 -- MTRef R1/LConn1
  Damper2/LConn1 -- R2/RConn1
  Damper2/RConn1 -- MTRef R2/LConn1
  Damper3/LConn1 -- L2/RConn1
  Damper3/RConn1 -- MTRef L2/LConn1
  Damper/LConn1 -- L1/RConn1
  Damper/RConn1 -- MTRef L1/LConn1

== system sm_car_/Vehicle/Vehicle/Chassis/Spring/Decoupled ==
  In Bus Element1 : Inport  PortName=Ctrl  Element=L1
  In Bus Element2 : Inport  PortName=Ctrl  Element=R1
  In Bus Element3 : Inport  PortName=Ctrl  Element=L2
  In Bus Element4 : Inport  PortName=Ctrl  Element=R2
  MTRef Heave A1 : fl_lib/Mechanical/Translational Elements/Mechanical Translational Reference
  MTRef Heave A2 : fl_lib/Mechanical/Translational Elements/Mechanical Translational Reference
  MTRef Roll A1 : fl_lib/Mechanical/Translational Elements/Mechanical Translational Reference
  MTRef Roll A2 : fl_lib/Mechanical/Translational Elements/Mechanical Translational Reference
  Spring A1 Heave : Subsystem  Variant=on  VariantControlMode=label  VariantControl=Variant1  LabelModeActiveChoice=Linear  mask(Variants for Spring){Spring=Spring.Axle1.Heave, VariantLabel=Spring.Axle1.Heave.class.Value}
      mask prompts: Spring "Spring Parameters"; VariantLabel "Variant Label"
      mask help: Select option and provide parameters for spring. Option is chosen by string provided in Variant Label. The parameters for the selected option is contained in Spring data structure.
      mask init:
      | curblk = gcb;
      | 
      | % Set variant for this block 
      | set_param(curblk,'LabelModeActiveChoice',VariantLabel);
      settings: AttributesFormatString=%<ActiveVariant>
      mask Display: disp(' ')
  Spring A1 Roll : Subsystem  Variant=on  VariantControlMode=label  VariantControl=Variant1  LabelModeActiveChoice=Linear  mask(Variants for Spring){Spring=Spring.Axle1.Roll, VariantLabel=Spring.Axle1.Roll.class.Value}
      mask prompts: Spring "Spring Parameters"; VariantLabel "Variant Label"
      mask help: Select option and provide parameters for spring. Option is chosen by string provided in Variant Label. The parameters for the selected option is contained in Spring data structure.
      mask init:
      | curblk = gcb;
      | 
      | % Set variant for this block 
      | set_param(curblk,'LabelModeActiveChoice',VariantLabel);
      settings: AttributesFormatString=%<ActiveVariant>
      mask Display: disp(' ')
  Spring A2 Heave : Subsystem  Variant=on  VariantControlMode=label  VariantControl=Variant1  LabelModeActiveChoice=Linear  mask(Variants for Spring){Spring=Spring.Axle2.Heave, VariantLabel=Spring.Axle2.Heave.class.Value}
      mask prompts: Spring "Spring Parameters"; VariantLabel "Variant Label"
      mask help: Select option and provide parameters for spring. Option is chosen by string provided in Variant Label. The parameters for the selected option is contained in Spring data structure.
      mask init:
      | curblk = gcb;
      | 
      | % Set variant for this block 
      | set_param(curblk,'LabelModeActiveChoice',VariantLabel);
      settings: AttributesFormatString=%<ActiveVariant>
      mask Display: disp(' ')
  Spring A2 Roll : Subsystem  Variant=on  VariantControlMode=label  VariantControl=Variant1  LabelModeActiveChoice=Linear  mask(Variants for Spring){Spring=Spring.Axle2.Roll, VariantLabel=Spring.Axle2.Roll.class.Value}
      mask prompts: Spring "Spring Parameters"; VariantLabel "Variant Label"
      mask help: Select option and provide parameters for spring. Option is chosen by string provided in Variant Label. The parameters for the selected option is contained in Spring data structure.
      mask init:
      | curblk = gcb;
      | 
      | % Set variant for this block 
      | set_param(curblk,'LabelModeActiveChoice',VariantLabel);
      settings: AttributesFormatString=%<ActiveVariant>
      mask Display: disp(' ')
  L1 : PMIOPort  Side=Left
  R1 : PMIOPort  Port=2  Side=Right
  L2 : PMIOPort  Port=3  Side=Left
  R2 : PMIOPort  Port=4  Side=Right
  Out Bus Element : Outport  VectorParamsAs1DForOutWhenUnconnected=off  PortName=meas  Element=L1
  Out Bus Element1 : Outport  VectorParamsAs1DForOutWhenUnconnected=off  PortName=meas  Element=R1
  Out Bus Element2 : Outport  VectorParamsAs1DForOutWhenUnconnected=off  PortName=meas  Element=L2
  Out Bus Element3 : Outport  VectorParamsAs1DForOutWhenUnconnected=off  PortName=meas  Element=R2
  wires:
  In Bus Element1/1 -> Spring A1 Heave/1("Ctrl ")
  Spring A1 Heave/1(" meas") -> Out Bus Element/1
  In Bus Element2/1 -> Spring A1 Roll/1("Ctrl ")
  Spring A1 Roll/1(" meas") -> Out Bus Element1/1
  In Bus Element3/1 -> Spring A2 Heave/1("Ctrl ")
  Spring A2 Heave/1(" meas") -> Out Bus Element2/1
  In Bus Element4/1 -> Spring A2 Roll/1("Ctrl ")
  Spring A2 Roll/1(" meas") -> Out Bus Element3/1
  connections:
  Spring A1 Roll/LConn1 -- R1/RConn1
  Spring A1 Roll/RConn1 -- MTRef Roll A1/LConn1
  Spring A2 Roll/LConn1 -- R2/RConn1
  Spring A2 Roll/RConn1 -- MTRef Roll A2/LConn1
  Spring A2 Heave/LConn1 -- L2/RConn1
  Spring A2 Heave/RConn1 -- MTRef Heave A2/LConn1
  Spring A1 Heave/LConn1 -- L1/RConn1
  Spring A1 Heave/RConn1 -- MTRef Heave A1/LConn1

== system sm_car_/Vehicle/Vehicle/Chassis/Spring/Independent ==
  In Bus Element1 : Inport  PortName=Ctrl  Element=L1
  In Bus Element2 : Inport  PortName=Ctrl  Element=R1
  In Bus Element3 : Inport  PortName=Ctrl  Element=L2
  In Bus Element4 : Inport  PortName=Ctrl  Element=R2
  MTRef L1 : fl_lib/Mechanical/Translational Elements/Mechanical Translational Reference
  MTRef L2 : fl_lib/Mechanical/Translational Elements/Mechanical Translational Reference
  MTRef R1 : fl_lib/Mechanical/Translational Elements/Mechanical Translational Reference
  MTRef R2 : fl_lib/Mechanical/Translational Elements/Mechanical Translational Reference
  Spring L1 : Subsystem  Variant=on  VariantControlMode=label  VariantControl=Variant1  LabelModeActiveChoice=Linear  mask(Variants for Spring){Spring=Spring.Axle1, VariantLabel=Spring.Axle1.class.Value}
      mask prompts: Spring "Spring Parameters"; VariantLabel "Variant Label"
      mask help: Select option and provide parameters for spring. Option is chosen by string provided in Variant Label. The parameters for the selected option is contained in Spring data structure.
      mask init:
      | curblk = gcb;
      | 
      | % Set variant for this block 
      | set_param(curblk,'LabelModeActiveChoice',VariantLabel);
      settings: AttributesFormatString=%<ActiveVariant>
      mask Display: disp(' ')
  Spring L2 : Subsystem  Variant=on  VariantControlMode=label  VariantControl=Variant1  LabelModeActiveChoice=Linear  mask(Variants for Spring){Spring=Spring.Axle2, VariantLabel=Spring.Axle2.class.Value}
      mask prompts: Spring "Spring Parameters"; VariantLabel "Variant Label"
      mask help: Select option and provide parameters for spring. Option is chosen by string provided in Variant Label. The parameters for the selected option is contained in Spring data structure.
      mask init:
      | curblk = gcb;
      | 
      | % Set variant for this block 
      | set_param(curblk,'LabelModeActiveChoice',VariantLabel);
      settings: AttributesFormatString=%<ActiveVariant>
      mask Display: disp(' ')
  Spring R1 : Subsystem  Variant=on  VariantControlMode=label  VariantControl=Variant1  LabelModeActiveChoice=Linear  mask(Variants for Spring){Spring=Spring.Axle1, VariantLabel=Spring.Axle1.class.Value}
      mask prompts: Spring "Spring Parameters"; VariantLabel "Variant Label"
      mask help: Select option and provide parameters for spring. Option is chosen by string provided in Variant Label. The parameters for the selected option is contained in Spring data structure.
      mask init:
      | curblk = gcb;
      | 
      | % Set variant for this block 
      | set_param(curblk,'LabelModeActiveChoice',VariantLabel);
      settings: AttributesFormatString=%<ActiveVariant>
      mask Display: disp(' ')
  Spring R2 : Subsystem  Variant=on  VariantControlMode=label  VariantControl=Variant1  LabelModeActiveChoice=Linear  mask(Variants for Spring){Spring=Spring.Axle2, VariantLabel=Spring.Axle2.class.Value}
      mask prompts: Spring "Spring Parameters"; VariantLabel "Variant Label"
      mask help: Select option and provide parameters for spring. Option is chosen by string provided in Variant Label. The parameters for the selected option is contained in Spring data structure.
      mask init:
      | curblk = gcb;
      | 
      | % Set variant for this block 
      | set_param(curblk,'LabelModeActiveChoice',VariantLabel);
      settings: AttributesFormatString=%<ActiveVariant>
      mask Display: disp(' ')
  L1 : PMIOPort  Side=Left
  R1 : PMIOPort  Port=2  Side=Right
  L2 : PMIOPort  Port=3  Side=Left
  R2 : PMIOPort  Port=4  Side=Right
  Out Bus Element : Outport  VectorParamsAs1DForOutWhenUnconnected=off  PortName=meas  Element=L1
  Out Bus Element1 : Outport  VectorParamsAs1DForOutWhenUnconnected=off  PortName=meas  Element=R1
  Out Bus Element2 : Outport  VectorParamsAs1DForOutWhenUnconnected=off  PortName=meas  Element=L2
  Out Bus Element3 : Outport  VectorParamsAs1DForOutWhenUnconnected=off  PortName=meas  Element=R2
  wires:
  In Bus Element1/1 -> Spring L1/1("Ctrl ")
  Spring L1/1(" meas") -> Out Bus Element/1
  In Bus Element2/1 -> Spring R1/1("Ctrl ")
  Spring R1/1(" meas") -> Out Bus Element1/1
  In Bus Element3/1 -> Spring L2/1("Ctrl ")
  Spring L2/1(" meas") -> Out Bus Element2/1
  In Bus Element4/1 -> Spring R2/1("Ctrl ")
  Spring R2/1(" meas") -> Out Bus Element3/1
  connections:
  Spring R1/LConn1 -- R1/RConn1
  Spring R1/RConn1 -- MTRef R1/LConn1
  Spring R2/LConn1 -- R2/RConn1
  Spring R2/RConn1 -- MTRef R2/LConn1
  Spring L2/LConn1 -- L2/RConn1
  Spring L2/RConn1 -- MTRef L2/LConn1
  Spring L1/LConn1 -- L1/RConn1
  Spring L1/RConn1 -- MTRef L1/LConn1
